simulink model "phase1_tmp36_faults"  (R2026a)
settings: Solver=VariableStepAuto  StopTime=600
settings Model: Creator=vedant  LastModifiedBy=vedant

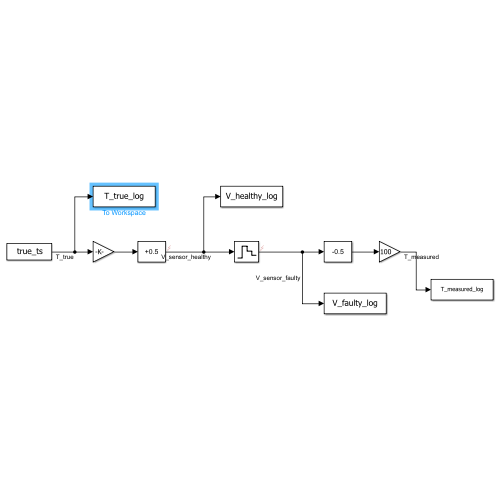
[thumbnail: Simulink's stored preview of the top-level diagram]
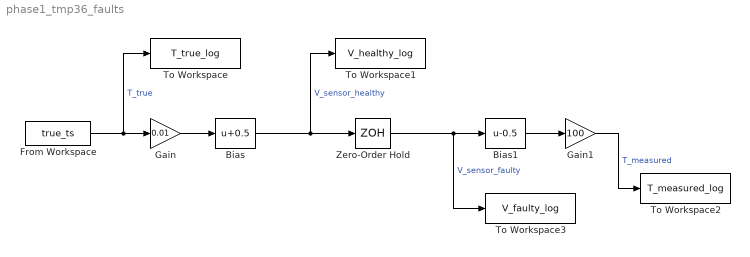
== system phase1_tmp36_faults ==
  Bias : Bias  Bias=0.5  SaturateOnIntegerOverflow=off
  Bias1 : Bias  Bias=-0.5  SaturateOnIntegerOverflow=off
  From Workspace : FromWorkspace  VariableName=true_ts
  Gain : Gain  Gain=0.01
  Gain1 : Gain  Gain=100
  To Workspace : ToWorkspace  VariableName=T_true_log  SaveFormat=Timeseries  SampleTime=-1
  To Workspace1 : ToWorkspace  VariableName=V_healthy_log  SaveFormat=Timeseries  SampleTime=-1
  To Workspace2 : ToWorkspace  VariableName=T_measured_log  SaveFormat=Timeseries  SampleTime=-1
  To Workspace3 : ToWorkspace  VariableName=V_faulty_log  SaveFormat=Timeseries  SampleTime=-1
  Zero-Order Hold : ZeroOrderHold  SampleTime=0.1
  wires:
  From Workspace/1 -> To Workspace/1, Gain/1  "T_true"
  Gain/1 -> Bias/1
  Bias/1 -> To Workspace1/1, Zero-Order Hold/1  "V_sensor_healthy"
  Bias1/1 -> Gain1/1
  Gain1/1 -> To Workspace2/1  "T_measured"
  Zero-Order Hold/1 -> Bias1/1, To Workspace3/1  "V_sensor_faulty"
